simulink model "modelo_eaf_dinamico"  (R2026a)
settings: Solver=ode45  StopTime=5
settings Model: Creator=dakra  LastModifiedBy=dakra

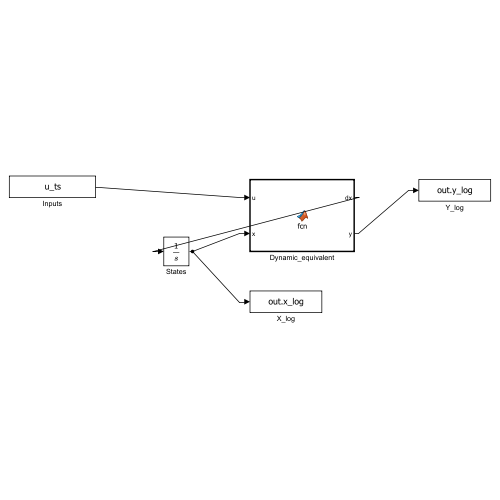
[thumbnail: Simulink's stored preview of the top-level diagram]
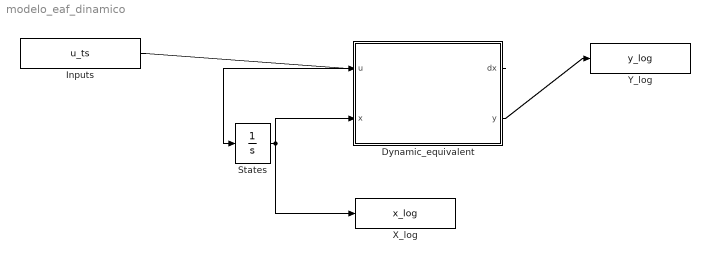
== system modelo_eaf_dinamico ==
  Dynamic_equivalent : MATLAB Function  TreatAsAtomicUnit=on
  Inputs : FromWorkspace  VariableName=u_ts
  States : Integrator  InitialCondition=[1;0]
  X_log : ToWorkspace  VariableName=x_log  SaveFormat=Timeseries  SampleTime=-1
  Y_log : ToWorkspace  VariableName=y_log  SaveFormat=Timeseries  SampleTime=-1
  wires:
  Inputs/1 -> Dynamic_equivalent/1(u)
  States/1 -> Dynamic_equivalent/2(x), X_log/1
  Dynamic_equivalent/1(dx) -> States/1
  Dynamic_equivalent/2(y) -> Y_log/1

== matlab function modelo_eaf_dinamico/Dynamic_equivalent ==
  data: dx output; u input; y output; x input
function [dx,y]=fcn(u,x)
p=u(1); q=u(2); en=u(3); vg=u(4); arc=u(5);
qgrid=abs(p)*tan(acos(0.95));
qref=en*min(0.277777777778,max(-0.277777777778,q-qgrid-0.166666666667));
qnet=q-0.166666666667-x(2);
vref=vg-0.005*p-0.143*qnet+arc;
dx=[(vref-x(1))/0.04;(qref-x(2))/0.08];
s=sqrt(p*p+qnet*qnet); pfout=abs(p)/max(s,1e-6);
y=[x(1);x(2);qnet;pfout];
end
